simulink subsystem "waypoint"  (R2026a)
settings: Solver=VariableStepAuto
libraries: simulink x2
settings Model: Creator=shrey  LastModifiedBy=shrey

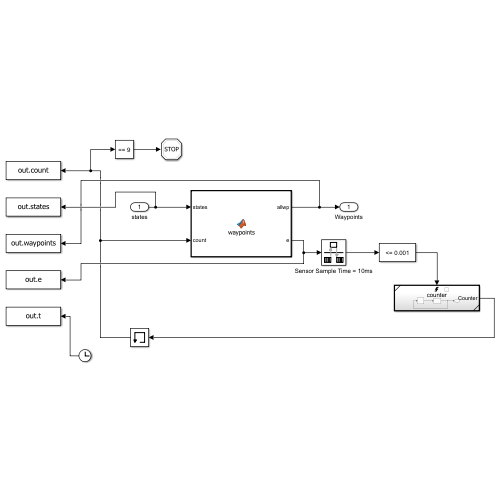
[thumbnail: Simulink's stored preview of the top-level diagram]
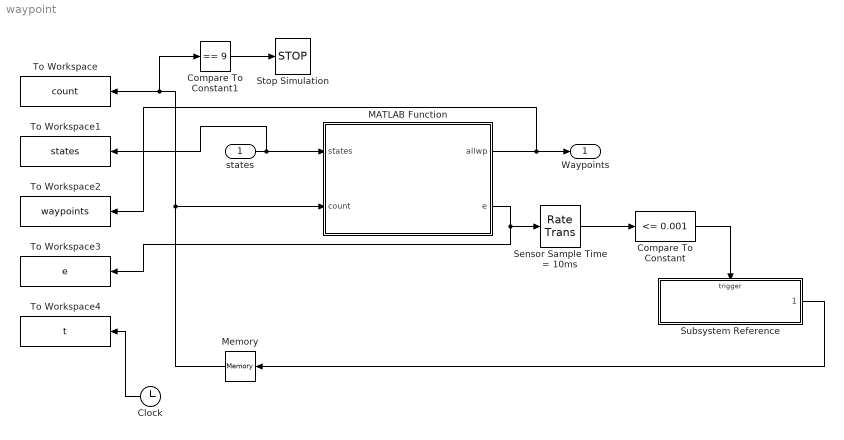
== system waypoint ==
  states : Inport
  Clock : Clock
  Compare To Constant : simulink/Logic and Bit Operations/Compare To Constant  relop=<=  const=0.001  OutDataTypeStr=boolean
  Compare To Constant1 : simulink/Logic and Bit Operations/Compare To Constant  relop===  const=9  OutDataTypeStr=boolean
  MATLAB Function : MATLAB Function  TreatAsAtomicUnit=on
  Memory : Memory  InheritSampleTime=on
  Sensor Sample Time = 10ms : RateTransition  OutPortSampleTime=0.01
  Stop Simulation : Stop
  Subsystem Reference : Subsystem  ReferencedSubsystem=counter
  To Workspace : ToWorkspace  VariableName=count  SaveFormat=Timeseries  SampleTime=-1
  To Workspace1 : ToWorkspace  VariableName=states  SaveFormat=Timeseries  SampleTime=-1
  To Workspace2 : ToWorkspace  VariableName=waypoints  SaveFormat=Timeseries  SampleTime=-1
  To Workspace3 : ToWorkspace  VariableName=e  SaveFormat=Timeseries  SampleTime=-1
  To Workspace4 : ToWorkspace  VariableName=t  SaveFormat=Timeseries  SampleTime=-1
  Waypoints : Outport
  wires:
  states/1 -> To Workspace1/1, MATLAB Function/1(states)
  MATLAB Function/1(allwp) -> To Workspace2/1, Waypoints/1
  MATLAB Function/2(e) -> To Workspace3/1, Sensor Sample Time = 10ms/1
  Sensor Sample Time = 10ms/1 -> Compare To Constant/1
  Compare To Constant/1 -> Subsystem Reference/Trigger
  Memory/1 -> MATLAB Function/2(count), Compare To Constant1/1, To Workspace/1
  Subsystem Reference/1 -> Memory/1
  Clock/1 -> To Workspace4/1
  Compare To Constant1/1 -> Stop Simulation/1

== matlab function waypoint/MATLAB Function ==
  data: states input; allwp output; count input; e output; p parameter
function [allwp,e] = waypoints(states,count,p)

allwp = zeros(12,1);
wp = zeros(3,1);
xi = states(1:3);
if count < 9
    wp = p.wp(:,uint8(count+1));
else
    wp(1) = 0;
    wp(2) = 0;
    wp(3) = 0;
end
e = norm(xi - wp);
allwp(1:3) = wp;
allwp(4:12) = 0;
